simulink library "ground_lib"  (R2018b)
settings: Solver=VariableStepAuto  StartTime=0.0  StopTime=10.0  RelTol=1e-3
undefined symbols (not defined in the file or in its folder): copter
libraries: axes_transformation_lib x2, flight_parameters_lib x2
settings Model: Creator=Ybeyer  LastModifiedBy=yannic
settings SFSimCC: SimUseLocalCustomCode=off
settings RTWCC: RTWUseLocalCustomCode=off
settings CodeAppCC: StateflowObjectComments=on

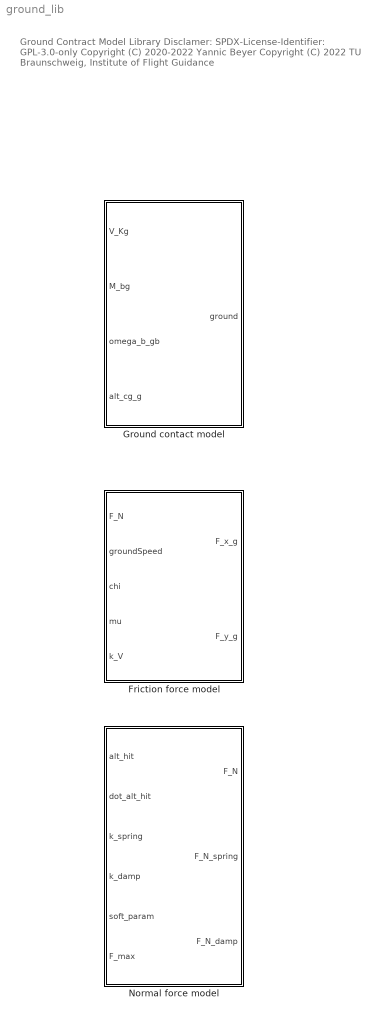
== system ground_lib ==
  note: Ground Contract Model Library
      |
      | Disclamer:
      | SPDX-License-Identifier: GPL-3.0-only
      |
      | Copyright (C) 2020-2022 Yannic Beyer
      | Copyright (C) 2022 TU Braunschweig, Institute of Flight Guidance
  Friction force model : MATLAB Function  TreatAsAtomicUnit=on
  Ground contact model : Subsystem  mask{m=copter.body.m, a_max=30, xyz_c_hit=copter.config.propPos_c, xyz_c_cg=copter.config.CoG_Pos_c, ground_softness_param=1e-5, k_h=1000, k_dot_h=100, mu=0.5, k_V=10}
      mask prompts: m "Aircraft mass, kg"; a_max "Maximum acceleration, m/s^2"; xyz_c_hit "Collision points (3xn) matrix for n collision points in body-fixed c frame, m"; xyz_c_cg "Center of gravity (3x1) vector in body-fixed c frame, m"; ground_softness_param "Ground softness parameter (>0), m. Close to zero means solid ground."; k_h "Ground spring stiffness, N/m"; k_dot_h "Ground damping, N.s/m"; mu "Ground friction coefficient, -"; k_V "Faktor for friction reduction (>0) at low speed, -. Large value for realistic results, small value to avoid shattering and slow simulation."
      mask DialogControl DescGroupVar Prompt: Ground contact model
      mask DialogControl DescTextVar Prompt: This block computes the forces and moments due to ground contact. Therefore, collision points of the vehicle as well as some parameters have to be defined.
  Normal force model : MATLAB Function  TreatAsAtomicUnit=on

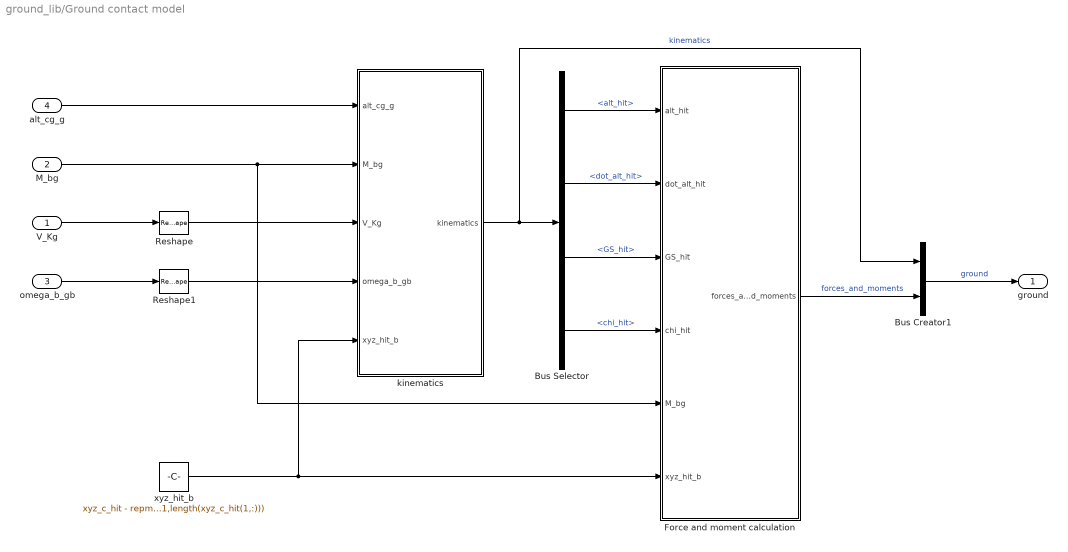
== system ground_lib/Ground contact model ==
  V_Kg : Inport
  M_bg : Inport  Port=2
  omega_b_gb : Inport  Port=3
  alt_cg_g : Inport  Port=4
  Bus Creator1 : BusCreator  Inputs=2
  Bus Selector : BusSelector  OutputSignals=alt_hit,dot_alt_hit,GS_hit,chi_hit
  Force and moment calculation : Subsystem
  Reshape : Reshape  OutputDimensionality=Column vector (2-D)
  Reshape1 : Reshape  OutputDimensionality=Column vector (2-D)
  kinematics : Subsystem
  xyz_hit_b : Constant  Value=xyz_c_hit - repmat(xyz_c_cg,1,length(xyz_c_hit(1,:)))
  ground : Outport
  wires:
  alt_cg_g/1 -> kinematics/1(alt_cg_g)
  Reshape1/1 -> kinematics/4(omega_b_gb)
  Bus Selector/1 -> Force and moment calculation/1(alt_hit)  "<alt_hit>"
  Bus Selector/3 -> Force and moment calculation/3(GS_hit)  "<GS_hit>"
  V_Kg/1 -> Reshape/1
  M_bg/1 -> kinematics/2(M_bg), Force and moment calculation/5(M_bg)
  Bus Selector/4 -> Force and moment calculation/4(chi_hit)  "<chi_hit>"
  xyz_hit_b/1 -> kinematics/5(xyz_hit_b), Force and moment calculation/6(xyz_hit_b)
  Force and moment calculation/1(forces_and_moments) -> Bus Creator1/2  "forces_and_moments"
  Bus Selector/2 -> Force and moment calculation/2(dot_alt_hit)  "<dot_alt_hit>"
  Reshape/1 -> kinematics/3(V_Kg)
  kinematics/1(kinematics) -> Bus Creator1/1, Bus Selector/1  "kinematics"
  Bus Creator1/1 -> ground/1  "ground"
  omega_b_gb/1 -> Reshape1/1

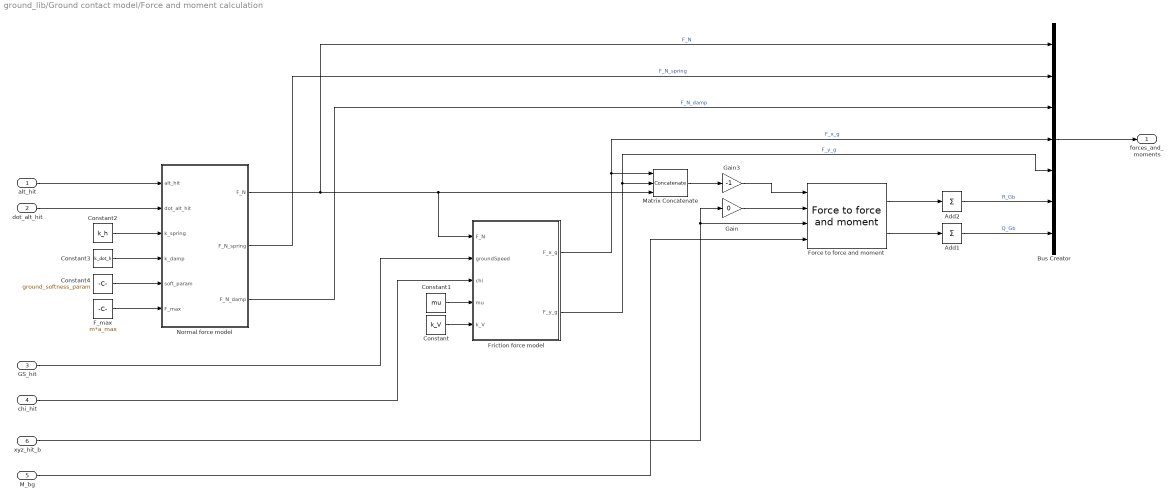
== system ground_lib/Ground contact model/Force and moment calculation ==
  alt_hit : Inport
  dot_alt_hit : Inport  Port=2
  GS_hit : Inport  Port=3
  chi_hit : Inport  Port=4
  M_bg : Inport  Port=5
  xyz_hit_b : Inport  Port=6
  Add1 : Sum  Inputs=+  CollapseMode=Specified dimension  CollapseDim=2
  Add2 : Sum  Inputs=+  CollapseMode=Specified dimension  CollapseDim=2
  Bus Creator : BusCreator  Inputs=7
  Constant : Constant  Value=k_V
  Constant1 : Constant  Value=mu
  Constant2 : Constant  Value=k_h
  Constant3 : Constant  Value=k_dot_h
  Constant4 : Constant  Value=ground_softness_param
  F_max : Constant  Value=m*a_max
  Force to force and moment : axes_transformation_lib/Force to force and moment  SystemSampleTime=-1
      settings: SourceProductName=LADAC
  Friction force model : MATLAB Function  TreatAsAtomicUnit=on
  Gain : Gain  Gain=0
  Gain3 : Gain  Gain=-1
  Matrix Concatenate : Concatenate  NumInputs=3  Mode=Multidimensional array
  Normal force model : MATLAB Function  TreatAsAtomicUnit=on
  forces_and_moments : Outport
  wires:
  Add1/1 -> Bus Creator/7  "Q_Gb"
  Add2/1 -> Bus Creator/6  "R_Gb"
  xyz_hit_b/1 -> Gain/1, Force to force and moment/3
  Normal force model/3(F_N_damp) -> Bus Creator/3  "F_N_damp"
  Normal force model/2(F_N_spring) -> Bus Creator/2  "F_N_spring"
  Constant/1 -> Friction force model/5(k_V)
  Constant1/1 -> Friction force model/4(mu)
  Friction force model/1(F_x_g) -> Matrix Concatenate/1, Bus Creator/4  "F_x_g"
  Friction force model/2(F_y_g) -> Matrix Concatenate/2, Bus Creator/5  "F_y_g"
  Gain/1 -> Force to force and moment/2
  Matrix Concatenate/1 -> Gain3/1
  Force to force and moment/1 -> Add2/1
  Force to force and moment/2 -> Add1/1
  Constant2/1 -> Normal force model/3(k_spring)
  Constant3/1 -> Normal force model/4(k_damp)
  Constant4/1 -> Normal force model/5(soft_param)
  dot_alt_hit/1 -> Normal force model/2(dot_alt_hit)
  Normal force model/1(F_N) -> Friction force model/1(F_N), Matrix Concatenate/3, Bus Creator/1  "F_N"
  M_bg/1 -> Force to force and moment/4
  Gain3/1 -> Force to force and moment/1
  F_max/1 -> Normal force model/6(F_max)
  alt_hit/1 -> Normal force model/1(alt_hit)
  GS_hit/1 -> Friction force model/2(groundSpeed)
  chi_hit/1 -> Friction force model/3(chi)
  Bus Creator/1 -> forces_and_moments/1

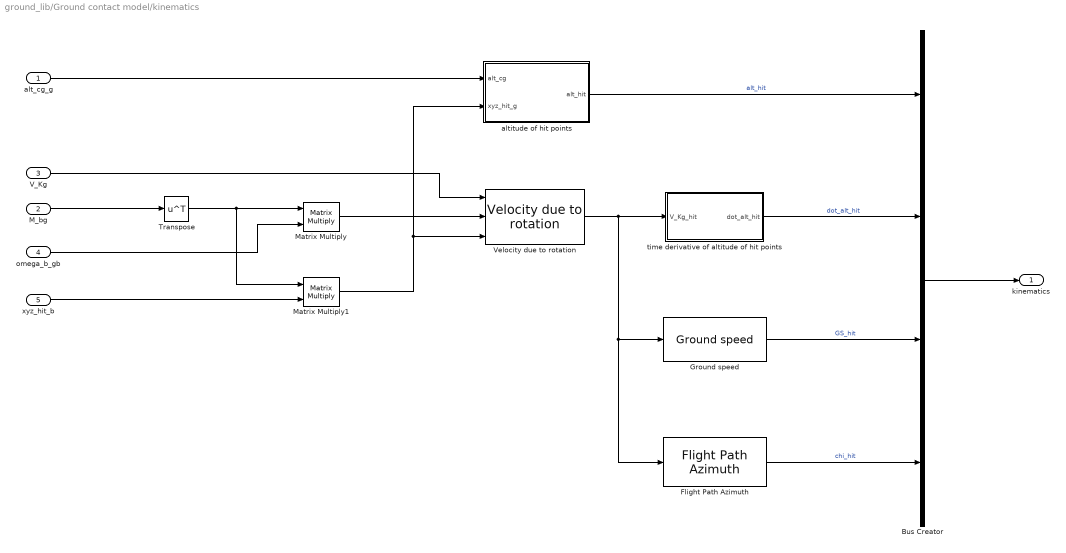
== system ground_lib/Ground contact model/kinematics ==
  alt_cg_g : Inport
  M_bg : Inport  Port=2
  V_Kg : Inport  Port=3
  omega_b_gb : Inport  Port=4
  xyz_hit_b : Inport  Port=5
  Bus Creator : BusCreator  Inputs=4
  Flight Path Azimuth : flight_parameters_lib/Flight Path Azimuth  SystemSampleTime=-1
      settings: SourceProductName=LADAC
  Ground speed : flight_parameters_lib/Ground speed  SystemSampleTime=-1
      settings: SourceProductName=LADAC
  Matrix Multiply : Product  Multiplication=Matrix(*)
  Matrix Multiply1 : Product  Multiplication=Matrix(*)
  Transpose : Math  Operator=transpose  SaturateOnIntegerOverflow=on
  Velocity due to rotation : axes_transformation_lib/Velocity due to rotation  SystemSampleTime=-1
      settings: SourceProductName=LADAC
  altitude of hit points : MATLAB Function  TreatAsAtomicUnit=on
  time derivative of altitude of hit points : MATLAB Function  TreatAsAtomicUnit=on
  kinematics : Outport
  wires:
  omega_b_gb/1 -> Matrix Multiply/2
  V_Kg/1 -> Velocity due to rotation/1
  alt_cg_g/1 -> altitude of hit points/1(alt_cg)
  M_bg/1 -> Transpose/1
  Matrix Multiply1/1 -> Velocity due to rotation/3, altitude of hit points/2(xyz_hit_g)
  Matrix Multiply/1 -> Velocity due to rotation/2
  Transpose/1 -> Matrix Multiply/1, Matrix Multiply1/1
  altitude of hit points/1(alt_hit) -> Bus Creator/1  "alt_hit"
  time derivative of altitude of hit points/1(dot_alt_hit) -> Bus Creator/2  "dot_alt_hit"
  xyz_hit_b/1 -> Matrix Multiply1/2
  Velocity due to rotation/1 -> Flight Path Azimuth/1, Ground speed/1, time derivative of altitude of hit points/1(V_Kg_hit)
  Ground speed/1 -> Bus Creator/3  "GS_hit"
  Flight Path Azimuth/1 -> Bus Creator/4  "chi_hit"
  Bus Creator/1 -> kinematics/1

== matlab function ground_lib/Normal force model ==
  data: alt_hit input; F_N output; dot_alt_hit input; k_spring input; k_damp input; soft_param input; F_max input; F_N_spring output; F_N_damp output
function [ F_N, F_N_spring, F_N_damp ] = fcn( alt_hit, ...
    dot_alt_hit, k_spring, k_damp, soft_param, F_max ) %#codegen
[ F_N, F_N_spring, F_N_damp ] = groundNormalForce( alt_hit, ...
    dot_alt_hit, k_spring, k_damp, soft_param, F_max );
end

== matlab function ground_lib/Friction force model ==
  data: F_N input; F_x_g output; groundSpeed input; chi input; mu input; k_V input; F_y_g output
function [ F_x_g, F_y_g ] = fcn( F_N, groundSpeed, chi, ...
    mu, k_V ) %#codegen
[ F_x_g, F_y_g ] = frictionModel( F_N, groundSpeed, chi, ...
    mu, k_V );
end

== matlab function ground_lib/Ground contact model/Force and moment calculation/Friction force model ==
  data: F_N input; F_x_g output; groundSpeed input; chi input; mu input; k_V input; F_y_g output
function [ F_x_g, F_y_g ] = fcn( F_N, groundSpeed, chi, ...
    mu, k_V ) %#codegen
[ F_x_g, F_y_g ] = frictionModel( F_N, groundSpeed, chi, ...
    mu, k_V );
end

== matlab function ground_lib/Ground contact model/Force and moment calculation/Normal force model ==
  data: alt_hit input; F_N output; dot_alt_hit input; k_spring input; k_damp input; soft_param input; F_max input; F_N_spring output; F_N_damp output
function [ F_N, F_N_spring, F_N_damp ] = fcn( alt_hit, ...
    dot_alt_hit, k_spring, k_damp, soft_param, F_max ) %#codegen
[ F_N, F_N_spring, F_N_damp ] = groundNormalForce( alt_hit, ...
    dot_alt_hit, k_spring, k_damp, soft_param, F_max );
end

== matlab function ground_lib/Ground contact model/kinematics/altitude of hit points ==
  data: alt_cg input; xyz_hit_g input; alt_hit output
function alt_hit = fcn( alt_cg, xyz_hit_g ) %#codegen
% compute altitude of hit points
num_hitpoints = length(xyz_hit_g(1,:));
alt_hit = [ -xyz_hit_g(3,:) + repmat(alt_cg,1,num_hitpoints) ];
end

== matlab function ground_lib/Ground contact model/kinematics/time derivative of altitude of hit points ==
  data: V_Kg_hit input; dot_alt_hit output
function dot_alt_hit = fcn( V_Kg_hit ) %#codegen
dot_alt_hit = - V_Kg_hit(3,:);
end
